simulink model "roll_pitch_yaw"  (R2024b)
settings: Solver=VariableStepAuto  StartTime=0.0  StopTime=10.0  FixedStep=0.001  RelTol=1e-3
libraries: sim3dlib x1, uavsim3dlib x1
settings Model: Creator=rupes  LastModifiedBy=rupes

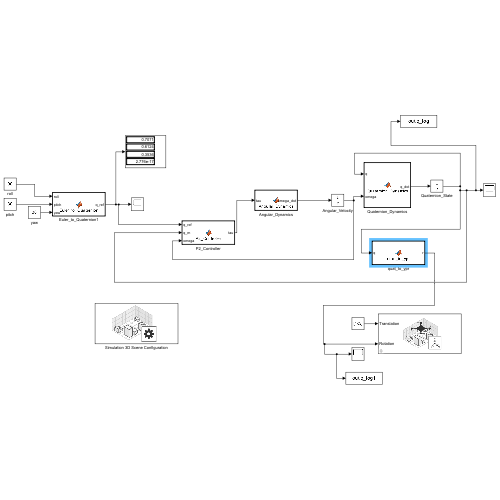
[thumbnail: Simulink's stored preview of the top-level diagram]
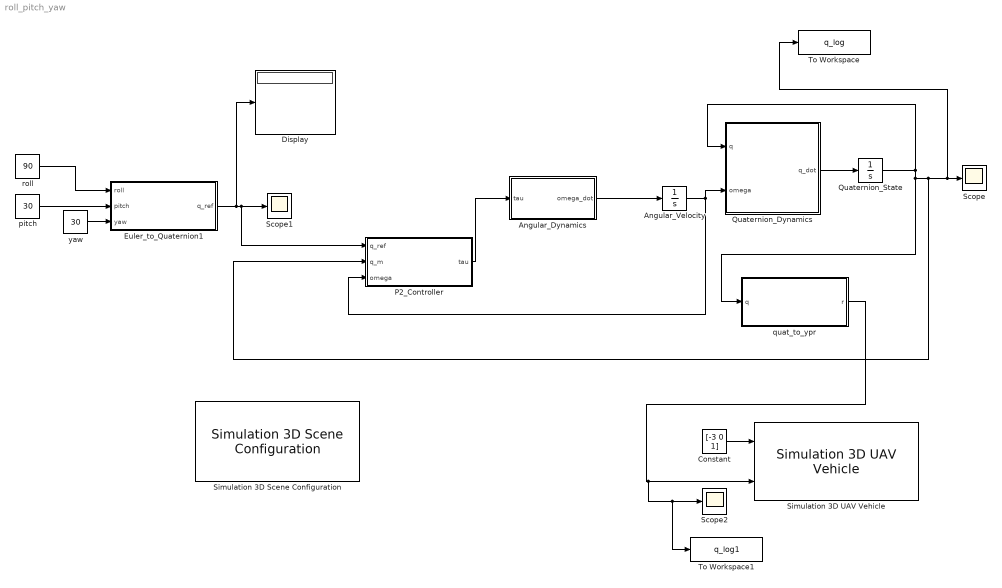
== system roll_pitch_yaw ==
  Angular_Dynamics : MATLAB Function  TreatAsAtomicUnit=on
  Angular_Velocity : Integrator  InitialCondition=[0; 0; 0]
  Constant : Constant  Value=[-3 0 1]
  Display : Display
  Euler_to_Quaternion1 : MATLAB Function  TreatAsAtomicUnit=on
  P2_Controller : MATLAB Function  TreatAsAtomicUnit=on
  Quaternion_Dynamics : MATLAB Function  TreatAsAtomicUnit=on
  Quaternion_State : Integrator  InitialCondition=[1; 0; 0; 0]
  Scope : Scope
  Scope1 : Scope
  Scope2 : Scope
  Simulation 3D Scene Configuration : sim3dlib/Simulation 3D Scene Configuration  Priority=0  ProjectFormat=Default Scenes  SceneDesc=US city block  ProjectName=C:\Program Files\MATLAB\R2024b\toolbox\shared\sim3d_projects\automotive_project_windows\UE\WindowsNoEditor\VehicleSimulation.exe  ScenePath=/Game/Maps/USCityBlock  EnableOpenDRIVE=off  vehTagList={'Custom';'Scene Origin';'SimulinkVehicle1'}  vehTag=Scene Origin  FreeCameraInitialTranslation=[0, 0, 0]  FreeCameraDefaultInitialTranslation=[-6, 0, 2]  FreeCameraInitialRotation=[0, 0, 0]  FreeCameraDefaultInitialRotation=[0, -15, 0]  OpVisEn=off  Ts=1/60  EnableWindow=on  EnableRemoteAccess=off  EnableWeather=off  SunAzimuth=90  SunAltitude=40.0  EnableGeospatialSun=off  Latitude=0  Longitude=0  Date=2023-01-01  Time=10:30:00  GeoTimeZone=-5.0  SunDaylightSaving=off  wind=1  clouds=10  EnableVolumetricClouds=off  CloudCoverage=0  CloudAltitude=6  fog=0  rain=0  RaindropsEffect=off  SnowDensity=0  EnableGeospatial=off  UseTrueOrigin=off  OriginHeight=200  OriginLatitude=40.744652  OriginLongitude=-73.988864  MapStyle=Aerial  AdditionalAssetIDs=[]  UseAdvancedSunSky=off  SolarTime=11  TimeZone=-5  Day=21  Month=9  Year=2022  UseDaylightSavingTime=on  DSTStartDay=10  DSTStartMonth=3  DSTEndDay=3  DSTEndMonth=11  DSTSwitchHour=2  sensorTag=MainCamera1  sensorId=1  sensorName=MainCamera1  mountLoc=Origin  offsetFlag=off  tmountOffset=[0, 0, 0]  rmountOffset=[0, 0, 0]  HorizontalResolution=1280  VerticalResolution=720  HorizontalFOV=60  mountPoint=[0 0 0]  mountOrientation=[0 0 0]  aMode=4  ID=1  GeoTrigger=Inactive
      settings: LibrarySourceBlock=uavsim3dlib/Simulation 3D Scene Configuration
  Simulation 3D UAV Vehicle : uavsim3dlib/Simulation 3D UAV Vehicle  Priority=-1  Mesh=Quadrotor  MeshPath=/MathWorksUAVContent/UAVs/HexaRotorUAV/HexaRotor.HexaRotor  Color=Black  ActorName=SimulinkVehicle1  UseGlobalFrame=off  InitialTranslation=[-3 0 1]  InitialRotation=[0 0 0]  InitialTranslationGlobal=[0 0 0]  InitialGeoOrigin=[0 0 0]  InitialRotationGlobal=[0 0 0]  SampleTime=-1  ActorType=SimulinkVehicle  ID=1  aMode=4  ActorTag=SimulinkVehicle1
  To Workspace : ToWorkspace  VariableName=q_log  SaveFormat=Timeseries  SampleTime=-1
  To Workspace1 : ToWorkspace  VariableName=q_log1  SaveFormat=Timeseries  SampleTime=-1
  pitch : Constant  Value=30
  quat_to_ypr : MATLAB Function  TreatAsAtomicUnit=on
  roll : Constant  Value=90
  yaw : Constant  Value=30
  wires:
  Angular_Velocity/1 -> P2_Controller/3(omega), Quaternion_Dynamics/2(omega)
  P2_Controller/1(tau) -> Angular_Dynamics/1(tau)
  Angular_Dynamics/1(omega_dot) -> Angular_Velocity/1
  Quaternion_Dynamics/1(q_dot) -> Quaternion_State/1
  Quaternion_State/1 -> quat_to_ypr/1(q), To Workspace/1, Scope/1, P2_Controller/2(q_m), Quaternion_Dynamics/1(q)
  Constant/1 -> Simulation 3D UAV Vehicle/1
  quat_to_ypr/1(r) -> To Workspace1/1, Scope2/1, Simulation 3D UAV Vehicle/2
  Euler_to_Quaternion1/1(q_ref) -> Scope1/1, P2_Controller/1(q_ref), Display/1
  roll/1 -> Euler_to_Quaternion1/1(roll)
  pitch/1 -> Euler_to_Quaternion1/2(pitch)
  yaw/1 -> Euler_to_Quaternion1/3(yaw)

== matlab function roll_pitch_yaw/Angular_Dynamics ==
  data: tau input; omega_dot output
function omega_dot = Angular_Dynamics(tau)

I = [1.4e-5  0       0;
     0       1.4e-5  0;
     0       0       2.2e-5];

omega_dot = I \ tau;

== matlab function roll_pitch_yaw/P2_Controller ==
  data: q_ref input; tau output; q_m input; omega input
function tau = P2_Controller(q_ref, q_m, omega)
%#codegen

Pq = 20;
Pomega = 4;

% Quaternion conjugate
% Quaternion format: [w x y z]
q_m_inv = [q_m(1);
          -q_m(2);
          -q_m(3);
          -q_m(4)];

% Quaternion error
q_error = quatMultiply(q_ref, q_m_inv);

% Vector part of quaternion error
q_error_vec = q_error(2:4);

% P2 controller
tau = Pq*q_error_vec - Pomega*omega;

end


function q = quatMultiply(a,b)
% Quaternion format: [w x y z]

q = zeros(4,1);

q(1) = a(1)*b(1) - a(2)*b(2) - a(3)*b(3) - a(4)*b(4);

q(2) = a(1)*b(2) + a(2)*b(1) + a(3)*b(4) - a(4)*b(3);

q(3) = a(1)*b(3) - a(2)*b(4) + a(3)*b(1) + a(4)*b(2);

q(4) = a(1)*b(4) + a(2)*b(3) - a(3)*b(2) + a(4)*b(1);

end

== matlab function roll_pitch_yaw/Quaternion_Dynamics ==
  data: q input; q_dot output; omega input
function q_dot = Quaternion_Dynamics(q, omega)

wx = omega(1);
wy = omega(2);
wz = omega(3);

Omega = [ 0   -wx  -wy  -wz;
          wx   0    wz  -wy;
          wy  -wz   0    wx;
          wz   wy  -wx   0  ];

q_dot = 0.5 * Omega * q;

== matlab function roll_pitch_yaw/quat_to_ypr ==
  data: q input; r output
function r = quat_to_ypr(q)
% Quaternion [w x y z] -> [yaw pitch roll]
% Output: [yaw; pitch; roll] in radians

% Quaternion components
w = q(1);
x = q(2);
y = q(3);
z = q(4);

% Normalize quaternion
n = sqrt(w*w + x*x + y*y + z*z);

if n > 0
    w = w/n;
    x = x/n;
    y = y/n;
    z = z/n;
end

% Roll
sinr = 2*(w*x + y*z);
cosr = 1 - 2*(x*x + y*y);
roll = atan2(sinr, cosr);

% Pitch
sinp = 2*(w*y - z*x);

if sinp > 1
    sinp = 1;
elseif sinp < -1
    sinp = -1;
end

pitch = asin(sinp);

% Yaw
siny = 2*(w*z + x*y);
cosy = 1 - 2*(y*y + z*z);
yaw = atan2(siny, cosy);

% Output: 3x1
r = [yaw; pitch; roll];

== matlab function roll_pitch_yaw/Euler_to_Quaternion1 ==
  data: roll input; q_ref output; pitch input; yaw input
function q_ref = Euler_to_Quaternion(roll, pitch, yaw)
%#codegen

r = roll*pi/180;
p = pitch*pi/180;
y = yaw*pi/180;

q0 = cos(r/2)*cos(p/2)*cos(y/2) ...
   + sin(r/2)*sin(p/2)*sin(y/2);

q1 = sin(r/2)*cos(p/2)*cos(y/2) ...
   - cos(r/2)*sin(p/2)*sin(y/2);

q2 = cos(r/2)*sin(p/2)*cos(y/2) ...
   + sin(r/2)*cos(p/2)*sin(y/2);

q3 = cos(r/2)*cos(p/2)*sin(y/2) ...
   - sin(r/2)*sin(p/2)*cos(y/2);

q_ref = [q0; q1; q2; q3];
end
